simulink model "afe"  (R2026a)
settings: Solver=ode23tb  StopTime=simlength  FixedStep=tc  MaxStep=glb_time.tc
values from neighbouring files (symbols this model uses):
  afe_ctrl = ctrl_afe_setup(glb_time.ts_afe, grid_emu.omega_grid_nom)    [init_model.m]
  afe_pwm_phase_shift_mod1 = 0    [init_model.m]
  CTRPIFF_CLIP_RELEASE = 0.001    [init_model.m]
  glb_time = timing_setup(fpwm_afe, trgo_afe, fpwm_inv, trgo_inv, fpwm_single_phase_inv, trgo_single_phase_inv, fpwm_dab, trgo_dab,      fpwm_psfbc, trgo_psfbc, fpwm_isop_rail, trgo_isop_rail, fpwm_cllc, trgo_cllc, t_measure, tc_factor, tc_decimation, delay_pwm, dead_time_afe,      dead_time_inv, dead_time_single_phase_inv, dead_time_dab, dead_time_psfbc, dead_time_isop_rail, dead_time_cllc)    [init_model.m]
  grid_emu = grid_three_phase_emulator('Dyn11', delta_star, grid_nominal_power, application_voltage, us1, us2, fgrid,                  eq_grid_inductance, eq_grid_resistance, eta, ucc, i1m, p_iron, n1, n2, core_area, core_length, mur,                  up_xi_pu_ref, up_eta_pu_ref, un_xi_pu_ref, un_eta_pu_ref)    [init_model.m]
  heatsink = liquid_cooled_plate_2kw_setup(weight, no_weight, cp_al, heat_capacity_hs, thermal_conductivity_al,      Rth_switch_HA, Rth_mosfet_HA, Rth_diode_HA, Tambient, DThs_init)    [init_model.m]
  ki_align = 18    [init_model.m]
  kp_align = 0.25    [init_model.m]
  lim_down_align = -0.05    [init_model.m]
  lim_up_align = 0.05    [init_model.m]
  psm_ctrl = ctrl_pmsm_setup(glb_time.ts_inv, psm.omega_bez, u_psm_scale, psm.Jm_norm)    [init_model.m]
  Tambient = 40    [init_model.m]
  time_gain_afe_module_1 = 1.0002    [init_model.m]
  time_gain_inv_module_2 = 1.001    [init_model.m]
  u_cm_comp_mod1 = 0    [init_model.m]
undefined symbols (not defined in the file or in its folder): hwdata, igbt, magnitude
libraries: fl_lib x166, nesl_utility x91, igbt_simple_2th_lib x6, single_phase_transformer_lib x3, discrete_time_low_pass_filter x1, threephase_inductor_lib x1, dclink_for_two_levels x1, three_phase_pwm_modulator x1, three_phase_voltage_with_frt_emulator x1
(part 3 of 7)

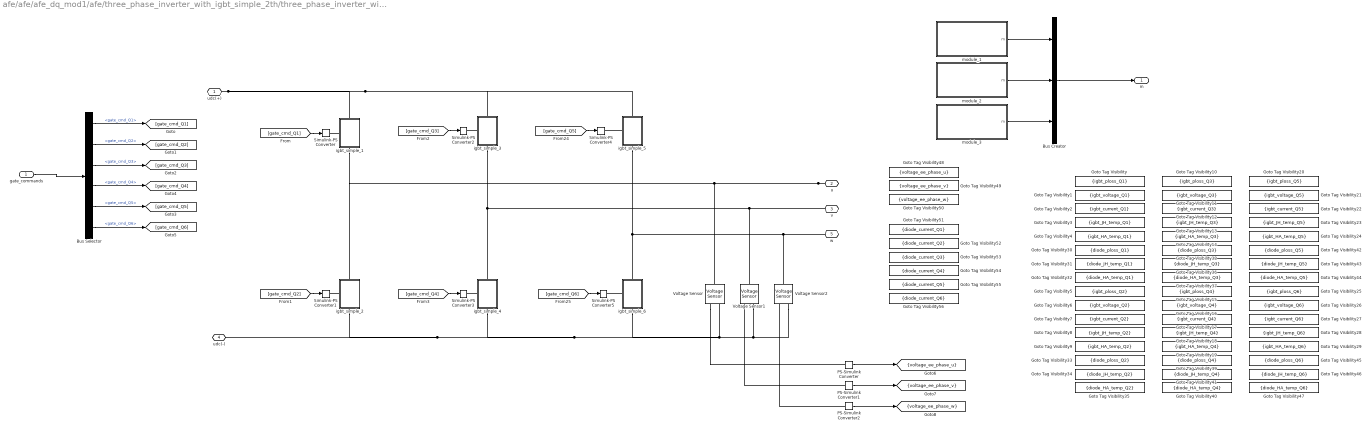
== system afe/afe/afe_dq_mod1/afe/three_phase_inverter_with_igbt_simple_2th/three_phase_inverter_with_igbt_simple_2th ==
  gate_commands : Inport
  Bus Creator : BusCreator  Inputs=3
  Bus Selector : BusSelector  OutputSignals=gate_cmd_Q1,gate_cmd_Q2,gate_cmd_Q3,gate_cmd_Q4,gate_cmd_Q5,gate_cmd_Q6
  Goto Tag Visibility : GotoTagVisibility  GotoTag=igbt_ploss_Q1
  Goto Tag Visibility1 : GotoTagVisibility  GotoTag=igbt_voltage_Q1
  Goto Tag Visibility10 : GotoTagVisibility  GotoTag=igbt_ploss_Q3
  Goto Tag Visibility11 : GotoTagVisibility  GotoTag=igbt_voltage_Q3
  Goto Tag Visibility12 : GotoTagVisibility  GotoTag=igbt_current_Q3
  Goto Tag Visibility13 : GotoTagVisibility  GotoTag=igbt_JH_temp_Q3
  Goto Tag Visibility14 : GotoTagVisibility  GotoTag=igbt_HA_temp_Q3
  Goto Tag Visibility15 : GotoTagVisibility  GotoTag=igbt_ploss_Q4
  Goto Tag Visibility16 : GotoTagVisibility  GotoTag=igbt_voltage_Q4
  Goto Tag Visibility17 : GotoTagVisibility  GotoTag=igbt_current_Q4
  Goto Tag Visibility18 : GotoTagVisibility  GotoTag=igbt_JH_temp_Q4
  Goto Tag Visibility19 : GotoTagVisibility  GotoTag=igbt_HA_temp_Q4
  Goto Tag Visibility2 : GotoTagVisibility  GotoTag=igbt_current_Q1
  Goto Tag Visibility20 : GotoTagVisibility  GotoTag=igbt_ploss_Q5
  Goto Tag Visibility21 : GotoTagVisibility  GotoTag=igbt_voltage_Q5
  Goto Tag Visibility22 : GotoTagVisibility  GotoTag=igbt_current_Q5
  Goto Tag Visibility23 : GotoTagVisibility  GotoTag=igbt_JH_temp_Q5
  Goto Tag Visibility24 : GotoTagVisibility  GotoTag=igbt_HA_temp_Q5
  Goto Tag Visibility25 : GotoTagVisibility  GotoTag=igbt_ploss_Q6
  Goto Tag Visibility26 : GotoTagVisibility  GotoTag=igbt_voltage_Q6
  Goto Tag Visibility27 : GotoTagVisibility  GotoTag=igbt_current_Q6
  Goto Tag Visibility28 : GotoTagVisibility  GotoTag=igbt_JH_temp_Q6
  Goto Tag Visibility29 : GotoTagVisibility  GotoTag=igbt_HA_temp_Q6
  Goto Tag Visibility3 : GotoTagVisibility  GotoTag=igbt_JH_temp_Q1
  Goto Tag Visibility30 : GotoTagVisibility  GotoTag=diode_ploss_Q1
  Goto Tag Visibility31 : GotoTagVisibility  GotoTag=diode_JH_temp_Q1
  Goto Tag Visibility32 : GotoTagVisibility  GotoTag=diode_HA_temp_Q1
  Goto Tag Visibility33 : GotoTagVisibility  GotoTag=diode_ploss_Q2
  Goto Tag Visibility34 : GotoTagVisibility  GotoTag=diode_JH_temp_Q2
  Goto Tag Visibility35 : GotoTagVisibility  GotoTag=diode_HA_temp_Q2
  Goto Tag Visibility36 : GotoTagVisibility  GotoTag=diode_JH_temp_Q3
  Goto Tag Visibility37 : GotoTagVisibility  GotoTag=diode_HA_temp_Q3
  Goto Tag Visibility38 : GotoTagVisibility  GotoTag=diode_ploss_Q3
  Goto Tag Visibility39 : GotoTagVisibility  GotoTag=diode_ploss_Q4
  Goto Tag Visibility4 : GotoTagVisibility  GotoTag=igbt_HA_temp_Q1
  Goto Tag Visibility40 : GotoTagVisibility  GotoTag=diode_HA_temp_Q4
  Goto Tag Visibility41 : GotoTagVisibility  GotoTag=diode_JH_temp_Q4
  Goto Tag Visibility42 : GotoTagVisibility  GotoTag=diode_ploss_Q5
  Goto Tag Visibility43 : GotoTagVisibility  GotoTag=diode_JH_temp_Q5
  Goto Tag Visibility44 : GotoTagVisibility  GotoTag=diode_HA_temp_Q5
  Goto Tag Visibility45 : GotoTagVisibility  GotoTag=diode_ploss_Q6
  Goto Tag Visibility46 : GotoTagVisibility  GotoTag=diode_JH_temp_Q6
  Goto Tag Visibility47 : GotoTagVisibility  GotoTag=diode_HA_temp_Q6
  Goto Tag Visibility48 : GotoTagVisibility  GotoTag=voltage_ee_phase_u
  Goto Tag Visibility49 : GotoTagVisibility  GotoTag=voltage_ee_phase_v
  Goto Tag Visibility5 : GotoTagVisibility  GotoTag=igbt_ploss_Q2
  Goto Tag Visibility50 : GotoTagVisibility  GotoTag=voltage_ee_phase_w
  Goto Tag Visibility51 : GotoTagVisibility  GotoTag=diode_current_Q1
  Goto Tag Visibility52 : GotoTagVisibility  GotoTag=diode_current_Q2
  Goto Tag Visibility53 : GotoTagVisibility  GotoTag=diode_current_Q3
  Goto Tag Visibility54 : GotoTagVisibility  GotoTag=diode_current_Q4
  Goto Tag Visibility55 : GotoTagVisibility  GotoTag=diode_current_Q5
  Goto Tag Visibility56 : GotoTagVisibility  GotoTag=diode_current_Q6
  Goto Tag Visibility6 : GotoTagVisibility  GotoTag=igbt_voltage_Q2
  Goto Tag Visibility7 : GotoTagVisibility  GotoTag=igbt_current_Q2
  Goto Tag Visibility8 : GotoTagVisibility  GotoTag=igbt_JH_temp_Q2
  Goto Tag Visibility9 : GotoTagVisibility  GotoTag=igbt_HA_temp_Q2
  PS-Simulink Converter : nesl_utility/PS-Simulink Converter  PhysicalDomain=network_engine_domain  SubClassName=ps_output  LeftPortType=input  RightPortType=output  PseudoPeriodic=off  Frequencies=[]  VectorFormat=1-D array  Unit=V  AffineConversion=off
  PS-Simulink Converter1 : nesl_utility/PS-Simulink Converter  PhysicalDomain=network_engine_domain  SubClassName=ps_output  LeftPortType=input  RightPortType=output  PseudoPeriodic=off  Frequencies=[]  VectorFormat=1-D array  Unit=V  AffineConversion=off
  PS-Simulink Converter2 : nesl_utility/PS-Simulink Converter  PhysicalDomain=network_engine_domain  SubClassName=ps_output  LeftPortType=input  RightPortType=output  PseudoPeriodic=off  Frequencies=[]  VectorFormat=1-D array  Unit=V  AffineConversion=off
  Simulink-PS Converter{,1..5} (6 alike) : nesl_utility/Simulink-PS Converter  PhysicalDomain=network_engine_domain  SubClassName=ps_input  LeftPortType=input  RightPortType=output  PseudoPeriodic=off  Frequencies=[]  NoiseDistribution=none  NoiseParameters=[]  Unit=V  AffineConversion=off  FilteringAndDerivatives=provide  SimscapeFilterOrder=1  InputFilterTimeConstant=0.001  UdotUserProvided=0
  Voltage Sensor : fl_lib/Electrical/Electrical Sensors/Voltage Sensor
  Voltage Sensor1 : fl_lib/Electrical/Electrical Sensors/Voltage Sensor
  Voltage Sensor2 : fl_lib/Electrical/Electrical Sensors/Voltage Sensor
  igbt_simple_1 : Subsystem
      settings: PortSchema="{\"entries\":[{\"content\":{\"sides\":[{\"content\":{\"connectorIds\":[\"LConn1\"]},\"type\":\"ConnectorPlacement.EquallySpacedRectSide\",\"uuid\":\"9277da8d-d460-43e6-8478-dd662f15d226\"},{\"content\":{\"connectorIds\":[],\"side\":\"RIGHT\"},\"type\":\"ConnectorPlacement.EquallySpacedRectSide\",\"uuid\":\"a7ece396-f1d9-4f4f-a05b-db1fc65d6e1d\"},{\"content\":{\"connectorIds\":[\"LConn2\"],\"side\":\"TOP\"},\"type\":\"ConnectorPlacement.EquallySpacedRectSide\",\"uuid\":\"fdd70777-e9cf-4317-afb6-cae87f75d5b0\"},{\"content\":{\"connectorIds\":[\"RConn1\"],\"side\":\"BOTTOM\"},\"type\":\"ConnectorPlacement.EquallySpacedRectSide\",\"uuid\":\"2353ed68-b1a1-4775-9ca9-31e268d5443b\"}]},\"type\":\"ConnectorPlacement.EquallySpacedConnector\",\"uuid\":\"d5479f4c-4e65-4791-adcb-73df11f88590\"}],\"packageUris\":[\"http://schema.mathworks.com/mf0/Connector/R2020b\"],\"version\":\"1.0\"}"
  igbt_simple_2 : Subsystem
      settings: PortSchema="{\"entries\":[{\"content\":{\"sides\":[{\"content\":{\"connectorIds\":[\"LConn1\"]},\"type\":\"ConnectorPlacement.EquallySpacedRectSide\",\"uuid\":\"9277da8d-d460-43e6-8478-dd662f15d226\"},{\"content\":{\"connectorIds\":[],\"side\":\"RIGHT\"},\"type\":\"ConnectorPlacement.EquallySpacedRectSide\",\"uuid\":\"a7ece396-f1d9-4f4f-a05b-db1fc65d6e1d\"},{\"content\":{\"connectorIds\":[\"LConn2\"],\"side\":\"TOP\"},\"type\":\"ConnectorPlacement.EquallySpacedRectSide\",\"uuid\":\"fdd70777-e9cf-4317-afb6-cae87f75d5b0\"},{\"content\":{\"connectorIds\":[\"RConn1\"],\"side\":\"BOTTOM\"},\"type\":\"ConnectorPlacement.EquallySpacedRectSide\",\"uuid\":\"2353ed68-b1a1-4775-9ca9-31e268d5443b\"}]},\"type\":\"ConnectorPlacement.EquallySpacedConnector\",\"uuid\":\"d5479f4c-4e65-4791-adcb-73df11f88590\"}],\"packageUris\":[\"http://schema.mathworks.com/mf0/Connector/R2020b\"],\"version\":\"1.0\"}"
  igbt_simple_3 : Subsystem
      settings: PortSchema="{\"entries\":[{\"content\":{\"sides\":[{\"content\":{\"connectorIds\":[\"LConn1\"]},\"type\":\"ConnectorPlacement.EquallySpacedRectSide\",\"uuid\":\"9277da8d-d460-43e6-8478-dd662f15d226\"},{\"content\":{\"connectorIds\":[],\"side\":\"RIGHT\"},\"type\":\"ConnectorPlacement.EquallySpacedRectSide\",\"uuid\":\"a7ece396-f1d9-4f4f-a05b-db1fc65d6e1d\"},{\"content\":{\"connectorIds\":[\"LConn2\"],\"side\":\"TOP\"},\"type\":\"ConnectorPlacement.EquallySpacedRectSide\",\"uuid\":\"fdd70777-e9cf-4317-afb6-cae87f75d5b0\"},{\"content\":{\"connectorIds\":[\"RConn1\"],\"side\":\"BOTTOM\"},\"type\":\"ConnectorPlacement.EquallySpacedRectSide\",\"uuid\":\"2353ed68-b1a1-4775-9ca9-31e268d5443b\"}]},\"type\":\"ConnectorPlacement.EquallySpacedConnector\",\"uuid\":\"d5479f4c-4e65-4791-adcb-73df11f88590\"}],\"packageUris\":[\"http://schema.mathworks.com/mf0/Connector/R2020b\"],\"version\":\"1.0\"}"
  igbt_simple_4 : Subsystem
      settings: PortSchema="{\"entries\":[{\"content\":{\"sides\":[{\"content\":{\"connectorIds\":[\"LConn1\"]},\"type\":\"ConnectorPlacement.EquallySpacedRectSide\",\"uuid\":\"9277da8d-d460-43e6-8478-dd662f15d226\"},{\"content\":{\"connectorIds\":[],\"side\":\"RIGHT\"},\"type\":\"ConnectorPlacement.EquallySpacedRectSide\",\"uuid\":\"a7ece396-f1d9-4f4f-a05b-db1fc65d6e1d\"},{\"content\":{\"connectorIds\":[\"LConn2\"],\"side\":\"TOP\"},\"type\":\"ConnectorPlacement.EquallySpacedRectSide\",\"uuid\":\"fdd70777-e9cf-4317-afb6-cae87f75d5b0\"},{\"content\":{\"connectorIds\":[\"RConn1\"],\"side\":\"BOTTOM\"},\"type\":\"ConnectorPlacement.EquallySpacedRectSide\",\"uuid\":\"2353ed68-b1a1-4775-9ca9-31e268d5443b\"}]},\"type\":\"ConnectorPlacement.EquallySpacedConnector\",\"uuid\":\"d5479f4c-4e65-4791-adcb-73df11f88590\"}],\"packageUris\":[\"http://schema.mathworks.com/mf0/Connector/R2020b\"],\"version\":\"1.0\"}"
  igbt_simple_5 : Subsystem
      settings: PortSchema="{\"entries\":[{\"content\":{\"sides\":[{\"content\":{\"connectorIds\":[\"LConn1\"]},\"type\":\"ConnectorPlacement.EquallySpacedRectSide\",\"uuid\":\"9277da8d-d460-43e6-8478-dd662f15d226\"},{\"content\":{\"connectorIds\":[],\"side\":\"RIGHT\"},\"type\":\"ConnectorPlacement.EquallySpacedRectSide\",\"uuid\":\"a7ece396-f1d9-4f4f-a05b-db1fc65d6e1d\"},{\"content\":{\"connectorIds\":[\"LConn2\"],\"side\":\"TOP\"},\"type\":\"ConnectorPlacement.EquallySpacedRectSide\",\"uuid\":\"fdd70777-e9cf-4317-afb6-cae87f75d5b0\"},{\"content\":{\"connectorIds\":[\"RConn1\"],\"side\":\"BOTTOM\"},\"type\":\"ConnectorPlacement.EquallySpacedRectSide\",\"uuid\":\"2353ed68-b1a1-4775-9ca9-31e268d5443b\"}]},\"type\":\"ConnectorPlacement.EquallySpacedConnector\",\"uuid\":\"d5479f4c-4e65-4791-adcb-73df11f88590\"}],\"packageUris\":[\"http://schema.mathworks.com/mf0/Connector/R2020b\"],\"version\":\"1.0\"}"
  igbt_simple_6 : Subsystem
      settings: PortSchema="{\"entries\":[{\"content\":{\"sides\":[{\"content\":{\"connectorIds\":[\"LConn1\"]},\"type\":\"ConnectorPlacement.EquallySpacedRectSide\",\"uuid\":\"9277da8d-d460-43e6-8478-dd662f15d226\"},{\"content\":{\"connectorIds\":[],\"side\":\"RIGHT\"},\"type\":\"ConnectorPlacement.EquallySpacedRectSide\",\"uuid\":\"a7ece396-f1d9-4f4f-a05b-db1fc65d6e1d\"},{\"content\":{\"connectorIds\":[\"LConn2\"],\"side\":\"TOP\"},\"type\":\"ConnectorPlacement.EquallySpacedRectSide\",\"uuid\":\"fdd70777-e9cf-4317-afb6-cae87f75d5b0\"},{\"content\":{\"connectorIds\":[\"RConn1\"],\"side\":\"BOTTOM\"},\"type\":\"ConnectorPlacement.EquallySpacedRectSide\",\"uuid\":\"2353ed68-b1a1-4775-9ca9-31e268d5443b\"}]},\"type\":\"ConnectorPlacement.EquallySpacedConnector\",\"uuid\":\"d5479f4c-4e65-4791-adcb-73df11f88590\"}],\"packageUris\":[\"http://schema.mathworks.com/mf0/Connector/R2020b\"],\"version\":\"1.0\"}"
  module_1 : Subsystem
  module_2 : Subsystem
  module_3 : Subsystem
  udc(+) : PMIOPort  Side=Left
  u : PMIOPort  Port=2  Side=Right
  v : PMIOPort  Port=3  Side=Right
  udc(-) : PMIOPort  Port=4  Side=Left
  w : PMIOPort  Port=5  Side=Right
  m : Outport
  tag scope: voltage_ee_phase_u=scoped, voltage_ee_phase_v=scoped, voltage_ee_phase_w=scoped
  wires:
  module_3/1(m) -> Bus Creator/3
  module_1/1(m) -> Bus Creator/1
  Bus Creator/1 -> m/1
  module_2/1(m) -> Bus Creator/2
  PS-Simulink Converter2/1 -> [voltage_ee_phase_w]
  PS-Simulink Converter1/1 -> [voltage_ee_phase_v]
  PS-Simulink Converter/1 -> [voltage_ee_phase_u]
  [gate_cmd_Q6] -> Simulink-PS Converter5/1
  [gate_cmd_Q5] -> Simulink-PS Converter4/1
  [gate_cmd_Q3] -> Simulink-PS Converter2/1
  [gate_cmd_Q4] -> Simulink-PS Converter3/1
  [gate_cmd_Q2] -> Simulink-PS Converter1/1
  [gate_cmd_Q1] -> Simulink-PS Converter/1
  gate_commands/1 -> Bus Selector/1
  Bus Selector/6 -> [gate_cmd_Q6]  "<gate_cmd_Q6>"
  Bus Selector/5 -> [gate_cmd_Q5]  "<gate_cmd_Q5>"
  Bus Selector/4 -> [gate_cmd_Q4]  "<gate_cmd_Q4>"
  Bus Selector/3 -> [gate_cmd_Q3]  "<gate_cmd_Q3>"
  Bus Selector/2 -> [gate_cmd_Q2]  "<gate_cmd_Q2>"
  Bus Selector/1 -> [gate_cmd_Q1]  "<gate_cmd_Q1>"
  connections:
  PS-Simulink Converter2/LConn1 -- Voltage Sensor2/RConn1
  PS-Simulink Converter1/LConn1 -- Voltage Sensor1/RConn1
  Voltage Sensor/RConn1 -- PS-Simulink Converter/LConn1
  w/RConn1 -- Voltage Sensor2/LConn1 -- igbt_simple_6/LConn2 -- igbt_simple_5/RConn1
  v/RConn1 -- Voltage Sensor1/LConn1 -- igbt_simple_4/LConn2 -- igbt_simple_3/RConn1
  Voltage Sensor1/RConn2 -- Voltage Sensor2/RConn2 -- Voltage Sensor/RConn2 -- igbt_simple_6/RConn1 -- igbt_simple_4/RConn1 -- igbt_simple_2/RConn1 -- udc(-)/RConn1
  igbt_simple_6/LConn1 -- Simulink-PS Converter5/RConn1
  igbt_simple_5/LConn1 -- Simulink-PS Converter4/RConn1
  igbt_simple_4/LConn1 -- Simulink-PS Converter3/RConn1
  igbt_simple_3/LConn1 -- Simulink-PS Converter2/RConn1
  igbt_simple_2/LConn1 -- Simulink-PS Converter1/RConn1
  igbt_simple_1/LConn1 -- Simulink-PS Converter/RConn1
  udc(+)/RConn1 -- igbt_simple_1/LConn2 -- igbt_simple_5/LConn2 -- igbt_simple_3/LConn2
  u/RConn1 -- Voltage Sensor/LConn1 -- igbt_simple_2/LConn2 -- igbt_simple_1/RConn1

== system afe/afe/afe_dq_mod1/AFE_control/afe_control/acquisitions/grid_phase_acquisition ==
  grid_phase : Inport
  Quantizer : Quantizer  QuantizationInterval=adc_quantization
  Unit Delay : UnitDelay  SampleTime=-1
  Zero-Order Hold : ZeroOrderHold  SampleTime=-1
  grid_phased : Outport
  wires:
  Zero-Order Hold/1 -> Quantizer/1
  Unit Delay/1 -> grid_phased/1
  grid_phase/1 -> Zero-Order Hold/1
  Quantizer/1 -> Unit Delay/1

== system afe/afe/afe_dq_mod1/AFE_control/afe_control/acquisitions/ig afe quantizzation and one step delay ==
  ig_abc_pu : Inport
  Demux1 : Demux  Outputs=3
  Mux1 : Mux  Inputs=3
  ig afe quantizzation and one step delay : Subsystem
  igd_abc_pu : Outport
  wires:
  Demux1/1 -> ig afe quantizzation and one step delay/1(ig_u_pu)
  Demux1/2 -> ig afe quantizzation and one step delay/2(ig_v_pu)
  ig_abc_pu/1 -> Demux1/1
  Mux1/1 -> igd_abc_pu/1
  Demux1/3 -> ig afe quantizzation and one step delay/3(ig_w_pu)
  ig afe quantizzation and one step delay/2(igd_v_pu) -> Mux1/2
  ig afe quantizzation and one step delay/1(igd_u_pu) -> Mux1/1
  ig afe quantizzation and one step delay/3(igd_w_pu) -> Mux1/3

== system afe/afe/afe_dq_mod1/AFE_control/afe_control/acquisitions/is afe quantizzation and one step delay ==
  is_abc_pu : Inport
  Demux : Demux  Outputs=3
  Mux : Mux  Inputs=3
  is afe quantizzation and one step delay : Subsystem
  isd_abc_pu : Outport
  wires:
  is afe quantizzation and one step delay/2(isd_v_pu) -> Mux/2
  is_abc_pu/1 -> Demux/1
  is afe quantizzation and one step delay/3(isd_w_pu) -> Mux/3
  is afe quantizzation and one step delay/1(isd_u_pu) -> Mux/1
  Demux/1 -> is afe quantizzation and one step delay/1(is_u_pu)
  Mux/1 -> isd_abc_pu/1
  Demux/3 -> is afe quantizzation and one step delay/3(is_w_pu)
  Demux/2 -> is afe quantizzation and one step delay/2(is_v_pu)

== system afe/afe/afe_dq_mod1/AFE_control/afe_control/acquisitions/phase_compensation_1 ==
  local_time : Inport
  master_time : Inport  Port=2
  Zero-Order Hold : ZeroOrderHold  SampleTime=-1
  Zero-Order Hold1 : ZeroOrderHold  SampleTime=-1
  alignment_eval_afe1 : Subsystem
  y : Outport
  wires:
  local_time/1 -> Zero-Order Hold/1
  master_time/1 -> Zero-Order Hold1/1
  alignment_eval_afe1/1(dp) -> y/1
  Zero-Order Hold/1 -> alignment_eval_afe1/1(local_time)
  Zero-Order Hold1/1 -> alignment_eval_afe1/2(master_time)

== system afe/afe/afe_dq_mod1/AFE_control/afe_control/acquisitions/udc_acquisition ==
  udc_pu : Inport
  Quantizer : Quantizer  QuantizationInterval=adc_quantization
  Unit Delay : UnitDelay  SampleTime=-1
  Zero-Order Hold : ZeroOrderHold  SampleTime=-1
  udcd_pu : Outport
  wires:
  Quantizer/1 -> Unit Delay/1
  udc_pu/1 -> Zero-Order Hold/1
  Unit Delay/1 -> udcd_pu/1
  Zero-Order Hold/1 -> Quantizer/1

== system afe/afe/afe_dq_mod1/AFE_control/afe_control/acquisitions/ug afe quantizzation and one step delay ==
  ug_abc_pu : Inport
  Demux : Demux  Outputs=3
  Mux : Mux  Inputs=3
  ug afe quantizzation and one step delay : Subsystem
  ugd_abc_pu : Outport
  wires:
  ug afe quantizzation and one step delay/2(ugd_v_pu) -> Mux/2
  Demux/2 -> ug afe quantizzation and one step delay/2(ug_v_pu)
  Demux/3 -> ug afe quantizzation and one step delay/3(ug_w_pu)
  ug afe quantizzation and one step delay/1(ugd_u_pu) -> Mux/1
  Demux/1 -> ug afe quantizzation and one step delay/1(ug_u_pu)
  ug_abc_pu/1 -> Demux/1
  ug afe quantizzation and one step delay/3(ugd_w_pu) -> Mux/3
  Mux/1 -> ugd_abc_pu/1

== system afe/afe/afe_dq_mod1/AFE_control/afe_control/current_ctrl/current_transformation ==
  is_a_pu : Inport
  is_b_pu : Inport  Port=2
  is_c_pu : Inport  Port=3
  alphabeta2xieta : MATLAB Function  TreatAsAtomicUnit=on
  uvw2alphabeta : MATLAB Function  TreatAsAtomicUnit=on
  tag scope: id_eta_pu=scoped, id_xi_pu=scoped
  wires:
  is_c_pu/1 -> uvw2alphabeta/3(w)
  alphabeta2xieta/2(eta) -> [id_eta_pu]  "ieta_pu"
  alphabeta2xieta/1(xi) -> [id_xi_pu]  "ixi_pu"
  is_b_pu/1 -> uvw2alphabeta/2(v)
  uvw2alphabeta/2(beta) -> alphabeta2xieta/2(beta)  "ibeta_pu"
  uvw2alphabeta/1(alpha) -> alphabeta2xieta/1(alpha)  "ialpha_pu"
  [phase_grid_pll] -> alphabeta2xieta/3(gamma)
  is_a_pu/1 -> uvw2alphabeta/1(u)

== system afe/afe/afe_dq_mod1/AFE_control/afe_control/current_ctrl/dq_vector_pi ==
  id : Inport
  id_ref : Inport  Port=2
  iq : Inport  Port=3
  iq_ref : Inport  Port=4
  Sum1 : Sum  Inputs=|-+
  Sum2 : Sum  Inputs=|-+
  bounder1 : Subsystem
  bounder2 : Subsystem
  pi_d : Subsystem
  pi_q : Subsystem
  switch : Subsystem
  vector lenght : Subsystem
  md_sat : Outport
  mq_sat : Outport  Port=2
  wires:
  bounder2/2(clip) -> switch/2(clip 2)
  vector lenght/2(m) -> bounder1/3(m), bounder2/1(m)
  Sum2/1 -> pi_q/1(iq_tilde)
  pi_d/1(ud_out) -> vector lenght/1(md), bounder1/1(md)
  pi_q/1(Vqs_out) -> bounder2/3(mq), vector lenght/2(mq)
  vector lenght/1(m_1) -> bounder1/2(m_1), bounder2/2(m_1)
  switch/1(clip) -> pi_q/2(clip), pi_d/2(clip)
  iq/1 -> Sum2/1
  Sum1/1 -> pi_d/1(id_tilde)
  bounder1/2(clip) -> switch/1(clip 1)
  id/1 -> Sum1/1
  bounder1/1(md_sat) -> md_sat/1
  bounder2/1(mq_sat) -> mq_sat/1
  id_ref/1 -> Sum1/2
  iq_ref/1 -> Sum2/2

== system afe/afe/afe_dq_mod1/AFE_control/afe_control/current_ctrl/zero_current_ctrl ==
  ualpha_ctrl_afe : Inport
  ubeta_ctrl_afe : Inport  Port=2
  Bus Creator1 : BusCreator  Inputs=3
  iz : Subsystem
  zero_sequence_current_ctrl : Subsystem
  uabg_ctrl_out : Outport
  wires:
  Bus Creator1/1 -> uabg_ctrl_out/1
  ualpha_ctrl_afe/1 -> Bus Creator1/1  "ualpha_ctrl_afe"
  ubeta_ctrl_afe/1 -> Bus Creator1/2  "ubeta_ctrl_afe"
  iz/1(iz) -> zero_sequence_current_ctrl/1(iz)
  zero_sequence_current_ctrl/1(ugamma_afe) -> Bus Creator1/3  "ugamma_ctrl_afe"

== system afe/afe/afe_dq_mod1/AFE_control/afe_control/data_to_worspace_module_1/dq_pll ==
  Bus Creator1 : BusCreator  Inputs=8
  dqPLLs : Outport
  wires:
  [phase_grid_fht_simulink_pll] -> Bus Creator1/5  "phase_grid_fht_simulink_pll"
  [omega_grid_fht_simulink_pll] -> Bus Creator1/6  "omega_grid_fht_simulink_pll"
  [omega_grid_fhtsr_dqpll] -> Bus Creator1/8  "omega_grid_fhtsr_dqpll"
  [phase_grid_fhtsr_dqpll] -> Bus Creator1/7  "phase_grid_fhtsr_dqpll"
  [omega_grid_dqpll_ccaller] -> Bus Creator1/4  "omega_grid_dqpll_ccaller"
  [phase_grid_dqpll_ccaller] -> Bus Creator1/3  "phase_grid_dqpll_ccaller"
  [omega_grid_pu_dqpll] -> Bus Creator1/2  "omega_grid_pu_dqpll"
  [phase_grid_dqpll] -> Bus Creator1/1  "phase_grid_dqpll"
  Bus Creator1/1 -> dqPLLs/1

== system afe/afe/afe_dq_mod1/AFE_control/afe_control/data_to_worspace_module_1/pwr_meter ==
  Bus Creator1 : BusCreator  Inputs=4
  m_pwr_meter : Outport
  wires:
  [u_grid_pu_rms] -> Bus Creator1/2  "u_grid_pu_rms"
  Bus Creator1/1 -> m_pwr_meter/1
  [pwr_act_grid] -> Bus Creator1/3  "pwr_act_grid"
  [pwr_react_grid] -> Bus Creator1/4  "pwr_react_grid"
  [i_grid_pu_rms] -> Bus Creator1/1  "i_grid_pu_rms"

== system afe/afe/afe_dq_mod1/AFE_control/afe_control/grid_voltage_phase_lock_loops/FHT-PLL ==
  ug_abc_pu : Inport
  pll_stageA : Subsystem
  pll_stageB : Subsystem
  gamma_grid_fht_pll : Outport
  omega_grid_fht_pll : Outport  Port=2
  wires:
  ug_abc_pu/1 -> pll_stageA/2(ug_abc_pu)
  pll_stageB/2(omega_grid_ddsrf_pll) -> omega_grid_fht_pll/1
  pll_stageA/1(u_grid_xi) -> pll_stageB/1(u_grid_pos_xi)  "u_grid_pos_xi"
  pll_stageA/2(u_grid_eta) -> pll_stageB/2(u_grid_pos_eta)  "u_grid_pos_eta"
  pll_stageB/1(gamma_grid_ddsrf_pll) -> gamma_grid_fht_pll/1, pll_stageA/1(gamma_grid)

== system afe/afe/afe_dq_mod1/AFE_control/afe_control/grid_voltage_phase_lock_loops/FHT-PLL_simulink ==
  ug_abc_pu : Inport
  pll_stageA : Subsystem
  pll_stageB : Subsystem
  gamma_grid_fht_pll : Outport
  omega_grid_fht_pll : Outport  Port=2
  wires:
  pll_stageB/1(gamma_grid_ddsrf_pll) -> pll_stageA/1(gamma_grid), gamma_grid_fht_pll/1
  pll_stageA/2(u_grid_eta) -> pll_stageB/2(u_grid_pos_eta)  "u_grid_pos_eta"
  pll_stageA/1(u_grid_xi) -> pll_stageB/1(u_grid_pos_xi)  "u_grid_pos_xi"
  pll_stageB/2(omega_grid_ddsrf_pll) -> omega_grid_fht_pll/1
  ug_abc_pu/1 -> pll_stageA/2(ug_abc_pu)

== system afe/afe/afe_dq_mod1/AFE_control/afe_control/grid_voltage_phase_lock_loops/dq_pll ==
  ug_abc_pu : Inport
  Goto Tag Visibility29 : GotoTagVisibility  GotoTag=Vgrid_unorm_dqpll
  pll_stageA : Subsystem
  pll_stageB : Subsystem
  phase_grid_dqpll : Outport
  omega_grid_pu_dqpll : Outport  Port=2
  wires:
  pll_stageA/2(u_grid_pos_eta) -> pll_stageB/2(u_grid_pos_eta)  "u_grid_pos_eta"
  pll_stageB/1(phase_grid_pll) -> phase_grid_dqpll/1, pll_stageA/1(phase_grid)
  pll_stageA/1(u_grid_pos_xi) -> pll_stageB/1(u_grid_pos_xi)  "u_grid_pos_xi"
  pll_stageB/2(omega_grid_pu_pll) -> omega_grid_pu_dqpll/1
  ug_abc_pu/1 -> pll_stageA/2(ug_abc)

== system afe/afe/afe_dq_mod1/AFE_control/afe_control/grid_voltage_phase_lock_loops/dq_pll_ccaller ==
  ug_abc_pu : Inport
  Bus Selector : BusSelector  OutputSignals=omega_pu_hat,gamma_hat,u_grid_xi,u_grid_eta,dqpll_pll_state
  C Caller : CCaller  FunctionName=dqpll_grid_process_simulink  PortSpecificationStruct="%)30     .    N H   8    (     @         %    \"     8    !     0         %  0 \"0    $    _    07)G3F%M90  4&]R=$YA;64 4V-O<&4     26YD97@     5'EP90      4VEZ90      27-';&]B86P   X    P    !@    @    $          4    (     0    ,    !         !   P!O=70 #@   #     &    \"     0         !0    @    !     P    $         $  # &]U=  .    .     8    (    !          %    \"     $    &     0         0   ...(+3319 chars)"
  Constant : Constant  Value=glb_time.ts_afe
  Data Type Conversion{1..2,4..5} (4 alike) : DataTypeConversion  OutDataTypeStr=single  SaturateOnIntegerOverflow=off  RndMeth=Floor
  Data Type Conversion{6..10} (5 alike) : DataTypeConversion  OutDataTypeStr=double  SaturateOnIntegerOverflow=off  RndMeth=Floor
  Data Type Conversion3 : DataTypeConversion  OutDataTypeStr=uint8  SaturateOnIntegerOverflow=off  RndMeth=Floor
  Demux : Demux  Outputs=3
  Step : Step  Time=0.01  InitialValue=1  FinalValue=0
  first_harmonic_tracker : Scope  NumInputPorts=3
      settings: ActiveDisplayYMinimum=-1.7184470891952515  ActiveDisplayYMaximum=1.8384636640548706
  first_harmonic_tracker_phase_u : Subsystem
  first_harmonic_tracker_phase_v : Subsystem
  first_harmonic_tracker_phase_w : Subsystem
  gamma_hat : Outport  VectorParamsAs1DForOutWhenUnconnected=off
  omega_pu_hat : Outport  Port=2  VectorParamsAs1DForOutWhenUnconnected=off
  dqpll_uxi : Outport  Port=3  VectorParamsAs1DForOutWhenUnconnected=off
  dqpll_ueta : Outport  Port=4  VectorParamsAs1DForOutWhenUnconnected=off
  dqpll_state : Outport  Port=5  VectorParamsAs1DForOutWhenUnconnected=off
  wires:
  Step/1 -> Data Type Conversion3/1
  Constant/1 -> Data Type Conversion1/1
  Data Type Conversion3/1 -> C Caller/1
  Data Type Conversion2/1 -> C Caller/2
  Data Type Conversion4/1 -> C Caller/3
  Data Type Conversion5/1 -> C Caller/4
  Data Type Conversion1/1 -> C Caller/5
  C Caller/1 -> Bus Selector/1
  Bus Selector/1 -> Data Type Conversion6/1  "<omega_pu_hat>"
  Bus Selector/2 -> Data Type Conversion7/1  "<gamma_hat>"
  Bus Selector/3 -> Data Type Conversion8/1  "<u_grid_xi>"
  Bus Selector/4 -> Data Type Conversion9/1  "<u_grid_eta>"
  Bus Selector/5 -> Data Type Conversion10/1  "<dqpll_pll_state>"
  Data Type Conversion7/1 -> gamma_hat/1
  Data Type Conversion10/1 -> dqpll_state/1
  Data Type Conversion8/1 -> dqpll_uxi/1
  Data Type Conversion9/1 -> dqpll_ueta/1
  ug_abc_pu/1 -> Demux/1
  Demux/1 -> first_harmonic_tracker_phase_u/1(u)
  Demux/2 -> first_harmonic_tracker_phase_v/1(u)
  Demux/3 -> first_harmonic_tracker_phase_w/1(u)
  Data Type Conversion6/1 -> omega_pu_hat/1
  first_harmonic_tracker_phase_u/1(u_hat) -> first_harmonic_tracker/1, Data Type Conversion2/1  "tracker_phase_u"
  first_harmonic_tracker_phase_v/1(u_hat) -> first_harmonic_tracker/2, Data Type Conversion4/1  "tracker_phase_v"
  first_harmonic_tracker_phase_w/1(u_hat) -> first_harmonic_tracker/3, Data Type Conversion5/1  "tracker_phase_w"

== system afe/afe/afe_dq_mod1/AFE_control/afe_control/instantaneus_power/abc2alphabeta ==
  a : Inport
  b : Inport  Port=2
  c : Inport  Port=3
  Gain1 : Gain  Gain=-1/2
  Gain11 : Gain  Gain=-1/2
  Gain2 : Gain  Gain=0
  Gain3 : Gain  Gain=sqrt(3)/2
  Gain4 : Gain  Gain=-sqrt(3)/2
  Gain8 : Gain  Gain=2/3
  Gain9 : Gain  Gain=2/3
  Sum : Sum  Inputs=+++
  Sum1 : Sum  Inputs=+++
  "alpha " : Outport  VectorParamsAs1DForOutWhenUnconnected=off
  "beta " : Outport  Port=2  VectorParamsAs1DForOutWhenUnconnected=off
  wires:
  Gain3/1 -> Sum1/2
  Gain2/1 -> Sum1/1
  Gain11/1 -> Sum/2
  Gain4/1 -> Sum1/3
  Sum1/1 -> Gain9/1
  Gain8/1 -> "alpha "/1
  Sum/1 -> Gain8/1
  c/1 -> Gain4/1, Gain1/1
  Gain9/1 -> "beta "/1
  b/1 -> Gain3/1, Gain11/1
  Gain1/1 -> Sum/3
  a/1 -> Gain2/1, Sum/1

== system afe/afe/afe_dq_mod1/AFE_control/afe_control/instantaneus_power/abc2alphabeta  ==
  a : Inport
  b : Inport  Port=2
  c : Inport  Port=3
  Gain1 : Gain  Gain=-1/2
  Gain11 : Gain  Gain=-1/2
  Gain2 : Gain  Gain=0
  Gain3 : Gain  Gain=sqrt(3)/2
  Gain4 : Gain  Gain=-sqrt(3)/2
  Gain8 : Gain  Gain=2/3
  Gain9 : Gain  Gain=2/3
  Sum : Sum  Inputs=+++
  Sum1 : Sum  Inputs=+++
  "alpha " : Outport  VectorParamsAs1DForOutWhenUnconnected=off
  "beta " : Outport  Port=2  VectorParamsAs1DForOutWhenUnconnected=off
  wires:
  a/1 -> Sum/1, Gain2/1
  Gain2/1 -> Sum1/1
  Gain9/1 -> "beta "/1
  Gain11/1 -> Sum/2
  c/1 -> Gain1/1, Gain4/1
  Sum/1 -> Gain8/1
  Sum1/1 -> Gain9/1
  Gain1/1 -> Sum/3
  Gain3/1 -> Sum1/2
  Gain4/1 -> Sum1/3
  Gain8/1 -> "alpha "/1
  b/1 -> Gain11/1, Gain3/1

== system afe/afe/afe_dq_mod1/AFE_control/afe_control/instantaneus_power/moving_avarage_p ==
  in : Inport
  Gain : Gain  Gain=afe_ctrl.rms.n1-1
  Gain1 : Gain  Gain=1/afe_ctrl.rms.n1
  Sum : Sum  Inputs=|++
  Unit Delay : UnitDelay  SampleTime=-1
  out : Outport  VectorParamsAs1DForOutWhenUnconnected=off
  wires:
  Gain/1 -> Sum/2
  Gain1/1 -> out/1, Unit Delay/1
  in/1 -> Sum/1
  Unit Delay/1 -> Gain/1
  Sum/1 -> Gain1/1

== system afe/afe/afe_dq_mod1/AFE_control/afe_control/instantaneus_power/moving_avarage_q ==
  in : Inport
  Gain : Gain  Gain=afe_ctrl.rms.n1-1
  Gain1 : Gain  Gain=1/afe_ctrl.rms.n1
  Sum : Sum  Inputs=|++
  Unit Delay : UnitDelay  SampleTime=-1
  out : Outport  VectorParamsAs1DForOutWhenUnconnected=off
  wires:
  Sum/1 -> Gain1/1
  Unit Delay/1 -> Gain/1
  in/1 -> Sum/1
  Gain1/1 -> Unit Delay/1, out/1
  Gain/1 -> Sum/2

== system afe/afe/afe_dq_mod1/AFE_control/afe_control/instantaneus_power/rms ==
  In1 : Inport
  Gain : Gain  Gain=afe_ctrl.rms.n10-1
  Gain1 : Gain  Gain=1/afe_ctrl.rms.n10
  Math Function : Math  Operator=magnitude^2  SignedPower=on
  Sqrt : Sqrt
  Sum : Sum  Inputs=|++
  Unit Delay : UnitDelay  SampleTime=-1
  Out1 : Outport  VectorParamsAs1DForOutWhenUnconnected=off
  wires:
  In1/1 -> Math Function/1
  Sum/1 -> Gain1/1
  Gain1/1 -> Sqrt/1, Unit Delay/1
  Unit Delay/1 -> Gain/1
  Math Function/1 -> Sum/1
  Sqrt/1 -> Out1/1
  Gain/1 -> Sum/2

== system afe/afe/afe_dq_mod1/AFE_control/afe_control/instantaneus_power/rms1 ==
  In1 : Inport
  Gain : Gain  Gain=afe_ctrl.rms.n10-1
  Gain1 : Gain  Gain=1/afe_ctrl.rms.n10
  Math Function : Math  Operator=magnitude^2  SignedPower=on
  Sqrt : Sqrt
  Sum : Sum  Inputs=|++
  Unit Delay : UnitDelay  SampleTime=-1
  Out1 : Outport  VectorParamsAs1DForOutWhenUnconnected=off
  wires:
  Gain/1 -> Sum/2
  Sqrt/1 -> Out1/1
  Math Function/1 -> Sum/1
  Unit Delay/1 -> Gain/1
  Gain1/1 -> Unit Delay/1, Sqrt/1
  Sum/1 -> Gain1/1
  In1/1 -> Math Function/1

== system afe/afe/afe_dq_mod1/AFE_control/afe_control/instantaneus_power/rms2 ==
  In1 : Inport
  Gain : Gain  Gain=afe_ctrl.rms.n10-1
  Gain1 : Gain  Gain=1/afe_ctrl.rms.n10
  Math Function : Math  Operator=magnitude^2  SignedPower=on
  Sqrt : Sqrt
  Sum : Sum  Inputs=|++
  Unit Delay : UnitDelay  SampleTime=-1
  Out1 : Outport  VectorParamsAs1DForOutWhenUnconnected=off
  wires:
  In1/1 -> Math Function/1
  Sum/1 -> Gain1/1
  Gain1/1 -> Sqrt/1, Unit Delay/1
  Unit Delay/1 -> Gain/1
  Math Function/1 -> Sum/1
  Sqrt/1 -> Out1/1
  Gain/1 -> Sum/2

== system afe/afe/afe_dq_mod1/AFE_control/afe_control/instantaneus_power/rms3 ==
  In1 : Inport
  Gain : Gain  Gain=afe_ctrl.rms.n10-1
  Gain1 : Gain  Gain=1/afe_ctrl.rms.n10
  Math Function : Math  Operator=magnitude^2  SignedPower=on
  Sqrt : Sqrt
  Sum : Sum  Inputs=|++
  Unit Delay : UnitDelay  SampleTime=-1
  Out1 : Outport  VectorParamsAs1DForOutWhenUnconnected=off
  wires:
  Gain/1 -> Sum/2
  Sqrt/1 -> Out1/1
  Math Function/1 -> Sum/1
  Unit Delay/1 -> Gain/1
  Gain1/1 -> Unit Delay/1, Sqrt/1
  Sum/1 -> Gain1/1
  In1/1 -> Math Function/1

== system afe/afe/afe_dq_mod1/AFE_control/afe_control/instantaneus_power/rms4 ==
  In1 : Inport
  Gain : Gain  Gain=afe_ctrl.rms.n10-1
  Gain1 : Gain  Gain=1/afe_ctrl.rms.n10
  Math Function : Math  Operator=magnitude^2  SignedPower=on
  Sqrt : Sqrt
  Sum : Sum  Inputs=|++
  Unit Delay : UnitDelay  SampleTime=-1
  Out1 : Outport  VectorParamsAs1DForOutWhenUnconnected=off
  wires:
  In1/1 -> Math Function/1
  Sum/1 -> Gain1/1
  Gain1/1 -> Sqrt/1, Unit Delay/1
  Unit Delay/1 -> Gain/1
  Math Function/1 -> Sum/1
  Sqrt/1 -> Out1/1
  Gain/1 -> Sum/2

== system afe/afe/afe_dq_mod1/AFE_control/afe_control/instantaneus_power/rms5 ==
  In1 : Inport
  Gain : Gain  Gain=afe_ctrl.rms.n10-1
  Gain1 : Gain  Gain=1/afe_ctrl.rms.n10
  Math Function : Math  Operator=magnitude^2  SignedPower=on
  Sqrt : Sqrt
  Sum : Sum  Inputs=|++
  Unit Delay : UnitDelay  SampleTime=-1
  Out1 : Outport  VectorParamsAs1DForOutWhenUnconnected=off
  wires:
  Gain/1 -> Sum/2
  Sqrt/1 -> Out1/1
  Math Function/1 -> Sum/1
  Unit Delay/1 -> Gain/1
  Gain1/1 -> Unit Delay/1, Sqrt/1
  Sum/1 -> Gain1/1
  In1/1 -> Math Function/1

== system afe/afe/afe_dq_mod1/afe/three_phase_inverter_with_igbt_simple_2th/three_phase_inverter_with_igbt_simple_2th/igbt_simple_1 ==
  note: P_sw
  Capacitor : fl_lib/Electrical/Electrical Elements/Capacitor  c=Csnubber_m F  r=Rsnubber_m Ohm  g=0 1/Ohm  i_specify=off  i_priority=None  i=0 A  i_nominal_specify=off  i_nominal_value=1  i_nominal_unit=A  v_specify=off  v_priority=None  v=0 V  v_nominal_specify=off  v_nominal_value=1  v_nominal_unit=V  vc_specify=off  vc_priority=High  vc=0 V  vc_nominal_specify=off  vc_nominal_value=1  vc_nominal_unit=V
  IGBT_simple : Subsystem
      settings: PortSchema="{\"entries\":[{\"content\":{\"sides\":[{\"content\":{\"connectorIds\":[\"LConn1\"]},\"type\":\"ConnectorPlacement.EquallySpacedRectSide\",\"uuid\":\"c3d88d60-081d-4221-ab18-079856838dba\"},{\"content\":{\"side\":\"RIGHT\"},\"type\":\"ConnectorPlacement.EquallySpacedRectSide\",\"uuid\":\"76e7d76c-8b60-4107-8aac-a7654bd886e1\"},{\"content\":{\"connectorIds\":[\"LConn2\"],\"side\":\"TOP\"},\"type\":\"ConnectorPlacement.EquallySpacedRectSide\",\"uuid\":\"fbef57e1-7143-4076-ada8-0654b1d9ee0b\"},{\"content\":{\"connectorIds\":[\"RConn1\"],\"side\":\"BOTTOM\"},\"type\":\"ConnectorPlacement.EquallySpacedRectSide\",\"uuid\":\"f2fea5db-9515-452a-a480-7d54bae36c49\"}]},\"type\":\"ConnectorPlacement.EquallySpacedConnector\",\"uuid\":\"cddff0b8-236e-4840-ad87-03abcdd65fe7\"}],\"packageUris\":[\"http://schema.mathworks.com/mf0/Connector/R2020b\"],\"version\":\"1.0\"}"
  Voltage Sensor : fl_lib/Electrical/Electrical Sensors/Voltage Sensor
  uph : nesl_utility/PS-Simulink Converter  PhysicalDomain=network_engine_domain  SubClassName=ps_output  LeftPortType=input  RightPortType=output  PseudoPeriodic=off  Frequencies=[]  VectorFormat=1-D array  Unit=V  AffineConversion=off
  G : PMIOPort  Side=Left
  C : PMIOPort  Port=2  Side=Left
  E : PMIOPort  Port=3  Side=Right
  tag scope: igbt_voltage_Q1=scoped
  wires:
  uph/1 -> [igbt_voltage_Q1]  "uph"
  connections:
  G/RConn1 -- IGBT_simple/LConn1
  Voltage Sensor/RConn1 -- uph/LConn1
  Capacitor/LConn1 -- Voltage Sensor/LConn1 -- C/RConn1 -- IGBT_simple/LConn2
  Capacitor/RConn1 -- Voltage Sensor/RConn2 -- E/RConn1 -- IGBT_simple/RConn1

== system afe/afe/afe_dq_mod1/afe/three_phase_inverter_with_igbt_simple_2th/three_phase_inverter_with_igbt_simple_2th/igbt_simple_2 ==
  note: P_sw
  Capacitor : fl_lib/Electrical/Electrical Elements/Capacitor  c=Csnubber_m F  r=Rsnubber_m Ohm  g=0 1/Ohm  i_specify=off  i_priority=None  i=0 A  i_nominal_specify=off  i_nominal_value=1  i_nominal_unit=A  v_specify=off  v_priority=None  v=0 V  v_nominal_specify=off  v_nominal_value=1  v_nominal_unit=V  vc_specify=off  vc_priority=High  vc=0 V  vc_nominal_specify=off  vc_nominal_value=1  vc_nominal_unit=V
  IGBT_simple : Subsystem
      settings: PortSchema="{\"entries\":[{\"content\":{\"sides\":[{\"content\":{\"connectorIds\":[\"LConn1\"]},\"type\":\"ConnectorPlacement.EquallySpacedRectSide\",\"uuid\":\"c3d88d60-081d-4221-ab18-079856838dba\"},{\"content\":{\"side\":\"RIGHT\"},\"type\":\"ConnectorPlacement.EquallySpacedRectSide\",\"uuid\":\"76e7d76c-8b60-4107-8aac-a7654bd886e1\"},{\"content\":{\"connectorIds\":[\"LConn2\"],\"side\":\"TOP\"},\"type\":\"ConnectorPlacement.EquallySpacedRectSide\",\"uuid\":\"fbef57e1-7143-4076-ada8-0654b1d9ee0b\"},{\"content\":{\"connectorIds\":[\"RConn1\"],\"side\":\"BOTTOM\"},\"type\":\"ConnectorPlacement.EquallySpacedRectSide\",\"uuid\":\"f2fea5db-9515-452a-a480-7d54bae36c49\"}]},\"type\":\"ConnectorPlacement.EquallySpacedConnector\",\"uuid\":\"cddff0b8-236e-4840-ad87-03abcdd65fe7\"}],\"packageUris\":[\"http://schema.mathworks.com/mf0/Connector/R2020b\"],\"version\":\"1.0\"}"
  Voltage Sensor : fl_lib/Electrical/Electrical Sensors/Voltage Sensor
  uph : nesl_utility/PS-Simulink Converter  PhysicalDomain=network_engine_domain  SubClassName=ps_output  LeftPortType=input  RightPortType=output  PseudoPeriodic=off  Frequencies=[]  VectorFormat=1-D array  Unit=V  AffineConversion=off
  G : PMIOPort  Side=Left
  C : PMIOPort  Port=2  Side=Left
  E : PMIOPort  Port=3  Side=Right
  tag scope: igbt_voltage_Q2=scoped
  wires:
  uph/1 -> [igbt_voltage_Q2]  "uph"
  connections:
  IGBT_simple/RConn1 -- E/RConn1 -- Capacitor/RConn1 -- Voltage Sensor/RConn2
  C/RConn1 -- IGBT_simple/LConn2 -- Capacitor/LConn1 -- Voltage Sensor/LConn1
  Voltage Sensor/RConn1 -- uph/LConn1
  G/RConn1 -- IGBT_simple/LConn1

== system afe/afe/afe_dq_mod1/afe/three_phase_inverter_with_igbt_simple_2th/three_phase_inverter_with_igbt_simple_2th/igbt_simple_3 ==
  note: P_sw
  Capacitor : fl_lib/Electrical/Electrical Elements/Capacitor  c=Csnubber_m F  r=Rsnubber_m Ohm  g=0 1/Ohm  i_specify=off  i_priority=None  i=0 A  i_nominal_specify=off  i_nominal_value=1  i_nominal_unit=A  v_specify=off  v_priority=None  v=0 V  v_nominal_specify=off  v_nominal_value=1  v_nominal_unit=V  vc_specify=off  vc_priority=High  vc=0 V  vc_nominal_specify=off  vc_nominal_value=1  vc_nominal_unit=V
  IGBT_simple : Subsystem
      settings: PortSchema="{\"entries\":[{\"content\":{\"sides\":[{\"content\":{\"connectorIds\":[\"LConn1\"]},\"type\":\"ConnectorPlacement.EquallySpacedRectSide\",\"uuid\":\"c3d88d60-081d-4221-ab18-079856838dba\"},{\"content\":{\"side\":\"RIGHT\"},\"type\":\"ConnectorPlacement.EquallySpacedRectSide\",\"uuid\":\"76e7d76c-8b60-4107-8aac-a7654bd886e1\"},{\"content\":{\"connectorIds\":[\"LConn2\"],\"side\":\"TOP\"},\"type\":\"ConnectorPlacement.EquallySpacedRectSide\",\"uuid\":\"fbef57e1-7143-4076-ada8-0654b1d9ee0b\"},{\"content\":{\"connectorIds\":[\"RConn1\"],\"side\":\"BOTTOM\"},\"type\":\"ConnectorPlacement.EquallySpacedRectSide\",\"uuid\":\"f2fea5db-9515-452a-a480-7d54bae36c49\"}]},\"type\":\"ConnectorPlacement.EquallySpacedConnector\",\"uuid\":\"cddff0b8-236e-4840-ad87-03abcdd65fe7\"}],\"packageUris\":[\"http://schema.mathworks.com/mf0/Connector/R2020b\"],\"version\":\"1.0\"}"
  Voltage Sensor : fl_lib/Electrical/Electrical Sensors/Voltage Sensor
  uph : nesl_utility/PS-Simulink Converter  PhysicalDomain=network_engine_domain  SubClassName=ps_output  LeftPortType=input  RightPortType=output  PseudoPeriodic=off  Frequencies=[]  VectorFormat=1-D array  Unit=V  AffineConversion=off
  G : PMIOPort  Side=Left
  C : PMIOPort  Port=2  Side=Left
  E : PMIOPort  Port=3  Side=Right
  tag scope: igbt_voltage_Q3=scoped
  wires:
  uph/1 -> [igbt_voltage_Q3]  "uph"
  connections:
  G/RConn1 -- IGBT_simple/LConn1
  Voltage Sensor/RConn1 -- uph/LConn1
  Voltage Sensor/LConn1 -- Capacitor/LConn1 -- IGBT_simple/LConn2 -- C/RConn1
  Voltage Sensor/RConn2 -- Capacitor/RConn1 -- E/RConn1 -- IGBT_simple/RConn1

== system afe/afe/afe_dq_mod1/afe/three_phase_inverter_with_igbt_simple_2th/three_phase_inverter_with_igbt_simple_2th/igbt_simple_4 ==
  note: P_sw
  Capacitor : fl_lib/Electrical/Electrical Elements/Capacitor  c=Csnubber_m F  r=Rsnubber_m Ohm  g=0 1/Ohm  i_specify=off  i_priority=None  i=0 A  i_nominal_specify=off  i_nominal_value=1  i_nominal_unit=A  v_specify=off  v_priority=None  v=0 V  v_nominal_specify=off  v_nominal_value=1  v_nominal_unit=V  vc_specify=off  vc_priority=High  vc=0 V  vc_nominal_specify=off  vc_nominal_value=1  vc_nominal_unit=V
  IGBT_simple : Subsystem
      settings: PortSchema="{\"entries\":[{\"content\":{\"sides\":[{\"content\":{\"connectorIds\":[\"LConn1\"]},\"type\":\"ConnectorPlacement.EquallySpacedRectSide\",\"uuid\":\"c3d88d60-081d-4221-ab18-079856838dba\"},{\"content\":{\"side\":\"RIGHT\"},\"type\":\"ConnectorPlacement.EquallySpacedRectSide\",\"uuid\":\"76e7d76c-8b60-4107-8aac-a7654bd886e1\"},{\"content\":{\"connectorIds\":[\"LConn2\"],\"side\":\"TOP\"},\"type\":\"ConnectorPlacement.EquallySpacedRectSide\",\"uuid\":\"fbef57e1-7143-4076-ada8-0654b1d9ee0b\"},{\"content\":{\"connectorIds\":[\"RConn1\"],\"side\":\"BOTTOM\"},\"type\":\"ConnectorPlacement.EquallySpacedRectSide\",\"uuid\":\"f2fea5db-9515-452a-a480-7d54bae36c49\"}]},\"type\":\"ConnectorPlacement.EquallySpacedConnector\",\"uuid\":\"cddff0b8-236e-4840-ad87-03abcdd65fe7\"}],\"packageUris\":[\"http://schema.mathworks.com/mf0/Connector/R2020b\"],\"version\":\"1.0\"}"
  Voltage Sensor : fl_lib/Electrical/Electrical Sensors/Voltage Sensor
  uph : nesl_utility/PS-Simulink Converter  PhysicalDomain=network_engine_domain  SubClassName=ps_output  LeftPortType=input  RightPortType=output  PseudoPeriodic=off  Frequencies=[]  VectorFormat=1-D array  Unit=V  AffineConversion=off
  G : PMIOPort  Side=Left
  C : PMIOPort  Port=2  Side=Left
  E : PMIOPort  Port=3  Side=Right
  tag scope: igbt_voltage_Q4=scoped
  wires:
  uph/1 -> [igbt_voltage_Q4]  "uph"
  connections:
  IGBT_simple/RConn1 -- E/RConn1 -- Capacitor/RConn1 -- Voltage Sensor/RConn2
  C/RConn1 -- IGBT_simple/LConn2 -- Capacitor/LConn1 -- Voltage Sensor/LConn1
  Voltage Sensor/RConn1 -- uph/LConn1
  G/RConn1 -- IGBT_simple/LConn1

== system afe/afe/afe_dq_mod1/afe/three_phase_inverter_with_igbt_simple_2th/three_phase_inverter_with_igbt_simple_2th/igbt_simple_5 ==
  note: P_sw
  Capacitor : fl_lib/Electrical/Electrical Elements/Capacitor  c=Csnubber_m F  r=Rsnubber_m Ohm  g=0 1/Ohm  i_specify=off  i_priority=None  i=0 A  i_nominal_specify=off  i_nominal_value=1  i_nominal_unit=A  v_specify=off  v_priority=None  v=0 V  v_nominal_specify=off  v_nominal_value=1  v_nominal_unit=V  vc_specify=off  vc_priority=High  vc=0 V  vc_nominal_specify=off  vc_nominal_value=1  vc_nominal_unit=V
  IGBT_simple : Subsystem
      settings: PortSchema="{\"entries\":[{\"content\":{\"sides\":[{\"content\":{\"connectorIds\":[\"LConn1\"]},\"type\":\"ConnectorPlacement.EquallySpacedRectSide\",\"uuid\":\"c3d88d60-081d-4221-ab18-079856838dba\"},{\"content\":{\"side\":\"RIGHT\"},\"type\":\"ConnectorPlacement.EquallySpacedRectSide\",\"uuid\":\"76e7d76c-8b60-4107-8aac-a7654bd886e1\"},{\"content\":{\"connectorIds\":[\"LConn2\"],\"side\":\"TOP\"},\"type\":\"ConnectorPlacement.EquallySpacedRectSide\",\"uuid\":\"fbef57e1-7143-4076-ada8-0654b1d9ee0b\"},{\"content\":{\"connectorIds\":[\"RConn1\"],\"side\":\"BOTTOM\"},\"type\":\"ConnectorPlacement.EquallySpacedRectSide\",\"uuid\":\"f2fea5db-9515-452a-a480-7d54bae36c49\"}]},\"type\":\"ConnectorPlacement.EquallySpacedConnector\",\"uuid\":\"cddff0b8-236e-4840-ad87-03abcdd65fe7\"}],\"packageUris\":[\"http://schema.mathworks.com/mf0/Connector/R2020b\"],\"version\":\"1.0\"}"
  Voltage Sensor : fl_lib/Electrical/Electrical Sensors/Voltage Sensor
  uph : nesl_utility/PS-Simulink Converter  PhysicalDomain=network_engine_domain  SubClassName=ps_output  LeftPortType=input  RightPortType=output  PseudoPeriodic=off  Frequencies=[]  VectorFormat=1-D array  Unit=V  AffineConversion=off
  G : PMIOPort  Side=Left
  C : PMIOPort  Port=2  Side=Left
  E : PMIOPort  Port=3  Side=Right
  tag scope: igbt_voltage_Q5=scoped
  wires:
  uph/1 -> [igbt_voltage_Q5]  "uph"
  connections:
  G/RConn1 -- IGBT_simple/LConn1
  Voltage Sensor/RConn1 -- uph/LConn1
  Voltage Sensor/LConn1 -- Capacitor/LConn1 -- IGBT_simple/LConn2 -- C/RConn1
  Voltage Sensor/RConn2 -- Capacitor/RConn1 -- E/RConn1 -- IGBT_simple/RConn1

== system afe/afe/afe_dq_mod1/afe/three_phase_inverter_with_igbt_simple_2th/three_phase_inverter_with_igbt_simple_2th/igbt_simple_6 ==
  note: P_sw
  Capacitor : fl_lib/Electrical/Electrical Elements/Capacitor  c=Csnubber_m F  r=Rsnubber_m Ohm  g=0 1/Ohm  i_specify=off  i_priority=None  i=0 A  i_nominal_specify=off  i_nominal_value=1  i_nominal_unit=A  v_specify=off  v_priority=None  v=0 V  v_nominal_specify=off  v_nominal_value=1  v_nominal_unit=V  vc_specify=off  vc_priority=High  vc=0 V  vc_nominal_specify=off  vc_nominal_value=1  vc_nominal_unit=V
  IGBT_simple : Subsystem
      settings: PortSchema="{\"entries\":[{\"content\":{\"sides\":[{\"content\":{\"connectorIds\":[\"LConn1\"]},\"type\":\"ConnectorPlacement.EquallySpacedRectSide\",\"uuid\":\"c3d88d60-081d-4221-ab18-079856838dba\"},{\"content\":{\"side\":\"RIGHT\"},\"type\":\"ConnectorPlacement.EquallySpacedRectSide\",\"uuid\":\"76e7d76c-8b60-4107-8aac-a7654bd886e1\"},{\"content\":{\"connectorIds\":[\"LConn2\"],\"side\":\"TOP\"},\"type\":\"ConnectorPlacement.EquallySpacedRectSide\",\"uuid\":\"fbef57e1-7143-4076-ada8-0654b1d9ee0b\"},{\"content\":{\"connectorIds\":[\"RConn1\"],\"side\":\"BOTTOM\"},\"type\":\"ConnectorPlacement.EquallySpacedRectSide\",\"uuid\":\"f2fea5db-9515-452a-a480-7d54bae36c49\"}]},\"type\":\"ConnectorPlacement.EquallySpacedConnector\",\"uuid\":\"cddff0b8-236e-4840-ad87-03abcdd65fe7\"}],\"packageUris\":[\"http://schema.mathworks.com/mf0/Connector/R2020b\"],\"version\":\"1.0\"}"
  Voltage Sensor : fl_lib/Electrical/Electrical Sensors/Voltage Sensor
  uph : nesl_utility/PS-Simulink Converter  PhysicalDomain=network_engine_domain  SubClassName=ps_output  LeftPortType=input  RightPortType=output  PseudoPeriodic=off  Frequencies=[]  VectorFormat=1-D array  Unit=V  AffineConversion=off
  G : PMIOPort  Side=Left
  C : PMIOPort  Port=2  Side=Left
  E : PMIOPort  Port=3  Side=Right
  tag scope: igbt_voltage_Q6=scoped
  wires:
  uph/1 -> [igbt_voltage_Q6]  "uph"
  connections:
  IGBT_simple/RConn1 -- E/RConn1 -- Capacitor/RConn1 -- Voltage Sensor/RConn2
  C/RConn1 -- IGBT_simple/LConn2 -- Capacitor/LConn1 -- Voltage Sensor/LConn1
  Voltage Sensor/RConn1 -- uph/LConn1
  G/RConn1 -- IGBT_simple/LConn1
